simulink model "mini_cuboid_simscape_swingup_sim"  (R2024a)
settings: Solver=ode23tb  StartTime=0.0  StopTime=Trun  MaxStep=1e-3  RelTol=1e-3
values from neighbouring files (symbols this model uses):
  N = numel(torque)    [export_swingup.m]    (also in mini_cuboid_swingup_ini.m = round(Trun / Ts))
  param = get_parameter()    [mini_cuboid_swingup_ini.m]
  s = tfine/Trun    [mini_cuboid_swingup_ini.m]
  Ts = 1e-3    (= 0.001)    [mini_cuboid_swingup_ini.m]
  Z = null(Aeq)    [mini_cuboid_swingup_ini.m]
undefined symbols (not defined in the file or in its folder): X, Y
libraries: sm_lib x10, nesl_utility x6
settings Model: Creator=pichim  LastModifiedBy=pichim
settings OptimizationCC: DefaultParameterBehavior=Inlined  BufferReuse=off
settings DebuggingCC: InitInArrayFormatMsg=none

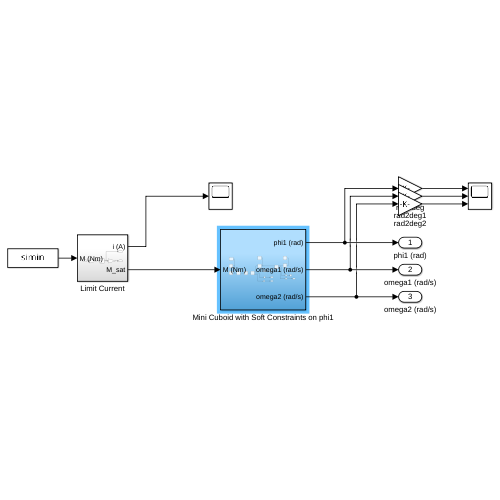
[thumbnail: Simulink's stored preview of the top-level diagram]
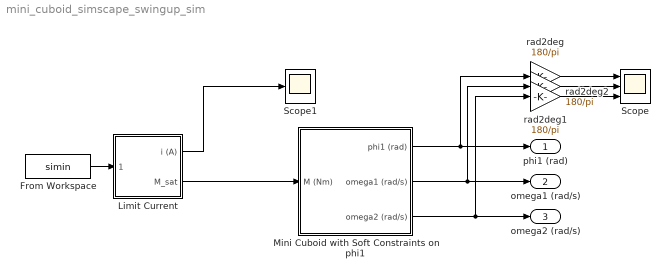
== system mini_cuboid_simscape_swingup_sim ==
  From Workspace : FromWorkspace  VariableName=simin  SampleTime=Ts  Interpolate=off  OutputAfterFinalValue=Holding final value
  Limit Current : Subsystem
  Mini Cuboid with Soft Constraints on phi1 : Subsystem
  Scope : Scope  NumInputPorts=3
  Scope1 : Scope
  rad2deg : Gain  Gain=180/pi
  rad2deg1 : Gain  Gain=180/pi
  rad2deg2 : Gain  Gain=180/pi
  phi1 (rad) : Outport
  omega1 (rad/s) : Outport  Port=2
  omega2 (rad/s) : Outport  Port=3
  wires:
  Limit Current/1(i (A)) -> Scope1/1
  Limit Current/2(M_sat) -> Mini Cuboid with Soft Constraints on phi1/1(M (Nm))
  Mini Cuboid with Soft Constraints on phi1/3(omega2 (rad/s)) -> rad2deg2/1, omega2 (rad/s)/1
  Mini Cuboid with Soft Constraints on phi1/2(omega1 (rad/s)) -> rad2deg1/1, omega1 (rad/s)/1
  Mini Cuboid with Soft Constraints on phi1/1(phi1 (rad)) -> phi1 (rad)/1, rad2deg/1
  From Workspace/1 -> Limit Current/1(M (Nm))
  rad2deg/1 -> Scope/1
  rad2deg1/1 -> Scope/2
  rad2deg2/1 -> Scope/3

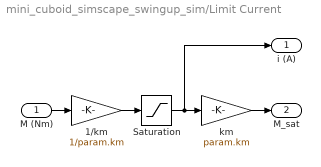
== system mini_cuboid_simscape_swingup_sim/Limit Current ==
  M (Nm) : Inport
  1/km : Gain  Gain=1/param.km
  Saturation : Saturate  UpperLimit=15  LowerLimit=-15
  km : Gain  Gain=param.km
  i (A) : Outport
  M_sat : Outport  Port=2
  wires:
  Saturation/1 -> i (A)/1, km/1
  1/km/1 -> Saturation/1
  M (Nm)/1 -> 1/km/1
  km/1 -> M_sat/1

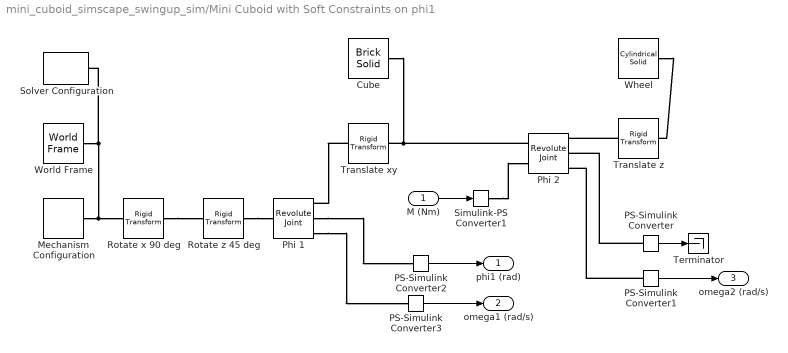
== system mini_cuboid_simscape_swingup_sim/Mini Cuboid with Soft Constraints on phi1 ==
  M (Nm) : Inport
  Cube : sm_lib/Body Elements/Brick Solid  BrickDimensions=[sqrt(2)*param.R sqrt(2)*param.R sqrt(2)*param.R/2]  BrickDimensionsUnits=m  ExportEntireGeometry=off  InertiaType=Custom  BasedOnType=Density  Density=1000  DensityUnits=kg/m^3  Mass=param.m  MassUnits=kg  CenterOfMass=[0 0 0]  CenterOfMassUnits=m  MomentsOfInertia=[0 0 param.J1]  MomentsOfInertiaUnits=kg*m^2  ProductsOfInertia=[0 0 0]  ProductsOfInertiaUnits=kg*m^2  GraphicType=FromGeometry  MarkerShape=Sphere  MarkerSize=10  GraphicVisPropType=SimpleVisualProperties  GraphicDiffuseColor=[0.0 0.4 0.8]  GraphicOpacity=1  GraphicSpecularColor=[0.5 0.5 0.5 1.0]  GraphicAmbientColor=[0.15 0.15 0.15 1.0]  GraphicEmissiveColor=[0.0 0.0 0.0 1.0]  GraphicShininess=75  DoExposeReferenceFrame=on  SerializedFrames=<Frames/>
  Mechanism Configuration : sm_lib/Utilities/Mechanism Configuration  UniformGravity=Constant  GravityVector=[0 0 -param.g]  GravityVectorUnits=m/s^2  LinearizationDelta=0.001  JointModeTransitionNonlinearIterations=2
  PS-Simulink Converter{,1..3} (4 alike) : nesl_utility/PS-Simulink Converter  PhysicalDomain=network_engine_domain  SubClassName=ps_output  LeftPortType=input  RightPortType=output  PseudoPeriodic=off  Frequencies=[]  VectorFormat=inherit  Unit=inherit  AffineConversion=off
  Phi 1 : sm_lib/Joints/Revolute Joint  JointMode=Normal  CompositeWrenchDir=FollowerOnBase  CompositeWrenchFrame=BaseFrame  SenseConstraintForce=off  SenseConstraintTorque=off  SenseTotalForce=off  SenseTotalTorque=off  PositionTargetSpecify=on  PositionTargetPriority=High  PositionTargetValue=phi1_0  PositionTargetValueUnits=rad  VelocityTargetSpecify=on  VelocityTargetPriority=High  VelocityTargetValue=omega1_0  VelocityTargetValueUnits=rad/s  EquilibriumPosition=0  EquilibriumPositionUnits=rad  SpringStiffness=0  SpringStiffnessUnits=N*m/rad  DampingCoefficient=0  DampingCoefficientUnits=N*m*s/rad  LowerLimitSpecify=on  LowerLimitBound=-pi/4  LowerLimitBoundUnits=rad  LowerLimitStiffness=100  LowerLimitStiffnessUnits=N*m/rad  LowerLimitDamping=1  LowerLimitDampingUnits=N*m*s/rad  LowerLimitTransitionRegionWidth=5e-4  LowerLimitTransitionRegionWidthUnits=rad  UpperLimitSpecify=on  UpperLimitBound=pi/4  UpperLimitBoundUnits=rad  UpperLimitStiffness=100  UpperLimitStiffnessUnits=N*m/rad  UpperLimitDamping=1  UpperLimitDampingUnits=N*m*s/rad  UpperLimitTransitionRegionWidth=5e-4  UpperLimitTransitionRegionWidthUnits=rad  TorqueActuationMode=NoTorque  MotionActuationMode=ComputedMotion  SensePosition=on  SenseVelocity=on  SenseAcceleration=off  SenseTorqueForce=off  SenseLowerLimitTorqueForce=off  SenseUpperLimitTorqueForce=off
  Phi 2 : sm_lib/Joints/Revolute Joint  JointMode=Normal  CompositeWrenchDir=FollowerOnBase  CompositeWrenchFrame=BaseFrame  SenseConstraintForce=off  SenseConstraintTorque=off  SenseTotalForce=off  SenseTotalTorque=off  PositionTargetSpecify=on  PositionTargetPriority=High  PositionTargetValue=phi2_0  PositionTargetValueUnits=rad  VelocityTargetSpecify=on  VelocityTargetPriority=High  VelocityTargetValue=omega2_0  VelocityTargetValueUnits=rad/s  EquilibriumPosition=0  EquilibriumPositionUnits=rad  SpringStiffness=0  SpringStiffnessUnits=N*m/rad  DampingCoefficient=0  DampingCoefficientUnits=N*m*s/rad  LowerLimitSpecify=off  LowerLimitBound=-90  LowerLimitBoundUnits=deg  LowerLimitStiffness=1e4  LowerLimitStiffnessUnits=N*m/deg  LowerLimitDamping=10  LowerLimitDampingUnits=N*m/(deg/s)  LowerLimitTransitionRegionWidth=0.1  LowerLimitTransitionRegionWidthUnits=deg  UpperLimitSpecify=off  UpperLimitBound=90  UpperLimitBoundUnits=deg  UpperLimitStiffness=1e4  UpperLimitStiffnessUnits=N*m/deg  UpperLimitDamping=10  UpperLimitDampingUnits=N*m/(deg/s)  UpperLimitTransitionRegionWidth=0.1  UpperLimitTransitionRegionWidthUnits=deg  TorqueActuationMode=InputTorque  MotionActuationMode=ComputedMotion  SensePosition=on  SenseVelocity=on  SenseAcceleration=off  SenseTorqueForce=off  SenseLowerLimitTorqueForce=off  SenseUpperLimitTorqueForce=off
  Rotate x 90 deg : sm_lib/Frames and Transforms/Rigid Transform  RotationMethod=RotationSequence  FollAlignAxisA=+X  BaseAlignAxisA=+Y  FollAlignAxisB=+Y  BaseAlignAxisB=+Z  RotationStandardAxis=+Z  RotationAngle=0  RotationAngleUnits=deg  RotationArbitraryAxis=[0 0 1]  RotationSequenceAxes=FollowerAxes  RotationSequence=ZYX  RotationSequenceAngles=[0 0 pi/2]  RotationSequenceAnglesUnits=rad  RotationMatrix=[1 0 0;0 1 0;0 0 1]  Quaternion=[1 0 0 0]  TranslationMethod=None  TranslationCartesianOffset=[0 0 0]  TranslationCartesianOffsetUnits=m  TranslationStandardAxis=+Z  TranslationStandardOffset=0  TranslationStandardOffsetUnits=m  TranslationROffset=0  TranslationROffsetUnits=m  TranslationThetaOffset=0  TranslationThetaOffsetUnits=deg  TranslationZOffset=0  TranslationZOffsetUnits=m
  Rotate z 45 deg : sm_lib/Frames and Transforms/Rigid Transform  RotationMethod=RotationSequence  FollAlignAxisA=+X  BaseAlignAxisA=+Y  FollAlignAxisB=+Y  BaseAlignAxisB=+Z  RotationStandardAxis=+Z  RotationAngle=0  RotationAngleUnits=deg  RotationArbitraryAxis=[0 0 1]  RotationSequenceAxes=FollowerAxes  RotationSequence=ZYX  RotationSequenceAngles=[pi/4 0 0]  RotationSequenceAnglesUnits=rad  RotationMatrix=[1 0 0;0 1 0;0 0 1]  Quaternion=[1 0 0 0]  TranslationMethod=None  TranslationCartesianOffset=[0 0 0]  TranslationCartesianOffsetUnits=m  TranslationStandardAxis=+Z  TranslationStandardOffset=0  TranslationStandardOffsetUnits=m  TranslationROffset=0  TranslationROffsetUnits=m  TranslationThetaOffset=0  TranslationThetaOffsetUnits=deg  TranslationZOffset=0  TranslationZOffsetUnits=m
  Simulink-PS Converter1 : nesl_utility/Simulink-PS Converter  PhysicalDomain=network_engine_domain  SubClassName=ps_input  LeftPortType=input  RightPortType=output  PseudoPeriodic=off  Frequencies=[]  NoiseDistribution=none  NoiseParameters=[]  Unit=1  AffineConversion=off  FilteringAndDerivatives=provide  SimscapeFilterOrder=1  InputFilterTimeConstant=0.001  UdotUserProvided=0
  Solver Configuration : nesl_utility/Solver Configuration  PhysicalDomain=network_engine_domain  SubClassName=solver  LeftPortType=input  RightPortType=generic  Tones=[]  Harmonics=[]  SimulateNoise=off  Profile=off  UseLocalSampling=off  EnableSwitchedLinearOptims=on  FrequencyDomain=off  UseCCode=off  RelTol=0.001  AbsTol=0.001  MinStep=1e-09  ToWorkspace=off  RevertToSquareIcSolve=off  NumHomotopyIterations=100  PhasorMode=off  PhasorModeNumHarmonics=1  ConsistencySolver=NEWTON_XTOL_AFTER_FTOL  IndexReductionMethod=DerivativeReplacement  DoDC=off  ResidualTolerance=1e-09  ConsistencyTolSource=GLOBAL  ConsistencyAbsTol=0.001  ConsistencyRelTol=0.001  ConsistencyTolFactor=0.001  UseLocalSolver=off  LocalSolverChoice=NE_BACKWARD_EULER_ADVANCER  ResolveIndetEquations=on  FunctionEvalNumThread=1  LocalSolverSampleTime=0.001  DoFixedCost=off  MaxNonlinIter=3  MaxModeIter=2  ComputeImpulses=off  ImpulseIterations=2  LinearAlgebra=auto  LinearAlgebraNumThread=0  EquationFormulation=NE_TIME_EF  DelaysMemoryBudget=1024  AutomaticFiltering=on  FilteringTimeConstant=0.001  PartitionStorageMethod=AS_NEEDED  PartitionMemoryBudget=1024  PartitionMethod=ROBUST  MultibodyUseLocalSolver=off  MultibodyLocalSolverChoice=ODE1  MultibodyLocalSolverSampleTime=0.001
  Terminator : Terminator
  Translate xy : sm_lib/Frames and Transforms/Rigid Transform  RotationMethod=None  FollAlignAxisA=+X  BaseAlignAxisA=+Y  FollAlignAxisB=+Y  BaseAlignAxisB=+Z  RotationStandardAxis=+Z  RotationAngle=0  RotationAngleUnits=deg  RotationArbitraryAxis=[0 0 1]  RotationSequenceAxes=FollowerAxes  RotationSequence=ZYX  RotationSequenceAngles=[0 0 0]  RotationSequenceAnglesUnits=rad  RotationMatrix=[1 0 0;0 1 0;0 0 1]  Quaternion=[1 0 0 0]  TranslationMethod=Cartesian  TranslationCartesianOffset=[sqrt(2)*param.R/2 sqrt(2)*param.R/2 0]  TranslationCartesianOffsetUnits=m  TranslationStandardAxis=+Z  TranslationStandardOffset=0  TranslationStandardOffsetUnits=m  TranslationROffset=0  TranslationROffsetUnits=m  TranslationThetaOffset=0  TranslationThetaOffsetUnits=deg  TranslationZOffset=0  TranslationZOffsetUnits=m
  Translate z : sm_lib/Frames and Transforms/Rigid Transform  RotationMethod=None  FollAlignAxisA=+X  BaseAlignAxisA=+Y  FollAlignAxisB=+Y  BaseAlignAxisB=+Z  RotationStandardAxis=+Z  RotationAngle=0  RotationAngleUnits=deg  RotationArbitraryAxis=[0 0 1]  RotationSequenceAxes=FollowerAxes  RotationSequence=ZYX  RotationSequenceAngles=[0 0 0]  RotationSequenceAnglesUnits=rad  RotationMatrix=[1 0 0;0 1 0;0 0 1]  Quaternion=[1 0 0 0]  TranslationMethod=Cartesian  TranslationCartesianOffset=[0 0 sqrt(2)*param.R/2/2+param.R/6/2]  TranslationCartesianOffsetUnits=m  TranslationStandardAxis=+Z  TranslationStandardOffset=0  TranslationStandardOffsetUnits=m  TranslationROffset=0  TranslationROffsetUnits=m  TranslationThetaOffset=0  TranslationThetaOffsetUnits=deg  TranslationZOffset=0  TranslationZOffsetUnits=m
  Wheel : sm_lib/Body Elements/Cylindrical Solid  CylinderRadius=param.R/sqrt(2)  CylinderRadiusUnits=m  CylinderLength=param.R/6  CylinderLengthUnits=m  ExportEntireGeometry=off  InertiaType=Custom  BasedOnType=Density  Density=1000  DensityUnits=kg/m^3  Mass=0  MassUnits=kg  CenterOfMass=[0 0 0]  CenterOfMassUnits=m  MomentsOfInertia=[0 0 param.J2]  MomentsOfInertiaUnits=kg*m^2  ProductsOfInertia=[0 0 0]  ProductsOfInertiaUnits=kg*m^2  GraphicType=FromGeometry  MarkerShape=Sphere  MarkerSize=10  GraphicVisPropType=SimpleVisualProperties  GraphicDiffuseColor=[1.0 0.9647059 0.2509804]  GraphicOpacity=1  GraphicSpecularColor=[0.5 0.5 0.5 1.0]  GraphicAmbientColor=[0.15 0.15 0.15 1.0]  GraphicEmissiveColor=[0.0 0.0 0.0 1.0]  GraphicShininess=75  DoExposeReferenceFrame=on  SerializedFrames=<Frames/>
  World Frame : sm_lib/Frames and Transforms/World Frame
  phi1 (rad) : Outport
  omega1 (rad/s) : Outport  Port=2
  omega2 (rad/s) : Outport  Port=3
  wires:
  M (Nm)/1 -> Simulink-PS Converter1/1
  PS-Simulink Converter2/1 -> phi1 (rad)/1
  PS-Simulink Converter/1 -> Terminator/1
  PS-Simulink Converter3/1 -> omega1 (rad/s)/1
  PS-Simulink Converter1/1 -> omega2 (rad/s)/1
  connections:
  PS-Simulink Converter1/LConn1 -- Phi 2/RConn3
  PS-Simulink Converter/LConn1 -- Phi 2/RConn2
  Simulink-PS Converter1/RConn1 -- Phi 2/LConn2
  Translate xy/LConn1 -- Phi 1/RConn1
  Rotate x 90 deg/RConn1 -- Rotate z 45 deg/LConn1
  Rotate z 45 deg/RConn1 -- Phi 1/LConn1
  World Frame/RConn1 -- Rotate x 90 deg/LConn1 -- Mechanism Configuration/RConn1 -- Solver Configuration/RConn1
  Cube/RConn1 -- Phi 2/LConn1 -- Translate xy/RConn1
  Translate z/LConn1 -- Phi 2/RConn1
  Wheel/RConn1 -- Translate z/RConn1
  Phi 1/RConn3 -- PS-Simulink Converter3/LConn1
  Phi 1/RConn2 -- PS-Simulink Converter2/LConn1
